simulink model "unit_can_sender"  (R2026b)
settings: Solver=FixedStepDiscrete  FixedStep=0.1  EnableMultiTasking=on
values from neighbouring files (symbols this model uses):
  BOOT_SEC = 10.0    [sign_detector.sldd]
  STALL_SEC = 1.0    [sign_detector.sldd]
libraries: raspberrypiCommlib x1
settings Model: DataDictionary=sign_detector.sldd  Creator=don  LastModifiedBy=don
settings SolverCC: PositivePriorityOrder=on
settings OptimizationCC: DifferentSizesBufferReuse=on  EfficientFloat2IntCast=on  EfficientTunableParamExpr=on  EnhancedBackFolding=on  LifeSpan=Inf  MaxStackSize=200000  OptimizationCustomize=off  OptimizeBlockOrder=speed  PassReuseOutputArgsAs=Individual arguments  UseDivisionForNetSlopeComputation=on
settings DebuggingCC: AlgebraicLoopMsg=error  ArtificialAlgebraicLoopMsg=error  AssertControl=DisableAll  BlockPriorityViolationMsg=error  BusObjectLabelMismatch=error  CheckMatrixSingularityMsg=error  InheritedTsInSrcMsg=error  IntegerOverflowMsg=error  IntegerSaturationMsg=error  ModelReferenceDataLoggingMessage=error  ModelReferenceIOMismatchMessage=error  NonBusSignalsTreatedAsBus=error  ParameterPrecisionLossMsg=error  ParameterTunabilityLossMsg=error  ParameterUnderflowMsg=error  ReadBeforeWriteMsg=EnableAllAsError  RootOutportRequireBusObject=error  SFcnCompatibilityMsg=error  SaveWithDisabledLinksMsg=error  SaveWithParameterizedLinksMsg=error  SigSpecEnsureSampleTimeMsg=error  SignalInfNanChecking=error  SignalLabelMismatchMsg=error  SignalRangeChecking=error  SolverPrmCheckMsg=error  StateNameClashWarn=warning  StrictBusMsg=ErrorOnBusTreatedAsVector  TasksWithSamePriorityMsg=error  UnconnectedInputMsg=error  UnconnectedLineMsg=error  UnconnectedOutputMsg=error  UnderSpecifiedDataTypeMsg=error  UniqueDataStoreMsg=error  UnknownTsInhSupMsg=error  UnnecessaryDatatypeConvMsg=warning  VariantConditionMismatch=error  VectorMatrixConversionMsg=error  WriteAfterReadMsg=EnableAllAsError  WriteAfterWriteMsg=EnableAllAsError
settings HardwareCC: ProdHWDeviceType=ARM Compatible->ARM Cortex-A (64-bit)  ProdLargestAtomicFloat=Double  ProdLargestAtomicInteger=LongLong  ProdLongLongMode=on
settings ModelReferenceCC: ModelReferenceNumInstancesAllowed=Single
settings SFSimCC: EnableRuntimeRecursion=off  MATLABDynamicMemAlloc=off
settings RTWCC: BuildConfiguration=Faster Runs  Description=Embedded Coder  HardwareBoard=Raspberry Pi (64bit)  SystemTargetFile=ert.tlc  TLCOptions="-aInlineSetEventsForThisBaseRateFcn=TLC_FALSE -aSuppressMultiTaskScheduler=TLC_FALSE  -aRateBasedStepFcn=0"  TargetLang=C++  TemplateMakefile=ert_default_tmf  Toolchain=GNU GCC RPIUtils
settings CodeAppCC: ForceParamTrailComments=on  IgnoreCustomStorageClasses=off  InsertBlockDesc=on  MATLABFcnDesc=on  MATLABSourceComments=on  OperatorAnnotations=on  ReqsInCode=on  SFDataObjDesc=on  SimulinkDataObjDesc=on  StateflowObjectComments=on
settings ERTTargetCC: CastingMode=Standards  CombineSignalStateStructs=on  EnableSignedLeftShifts=off  EnableSignedRightShifts=off  ExtModeIntrfLevel=Level2 - Open  ExtModeMexFile=ext_xcp  ExtModeStaticAlloc=on  GenerateSharedConstants=off  ParenthesesLevel=Standards  PreserveExpressionOrder=on  SubcomponentCodeInterfacePackaging=Nonreusable function  SupportNonFinite=off  SupportVariableSizeSignals=on  SuppressErrorStatus=on  TargetLangStandard=C++11 (ISO)  UtilityFuncGeneration=Shared location

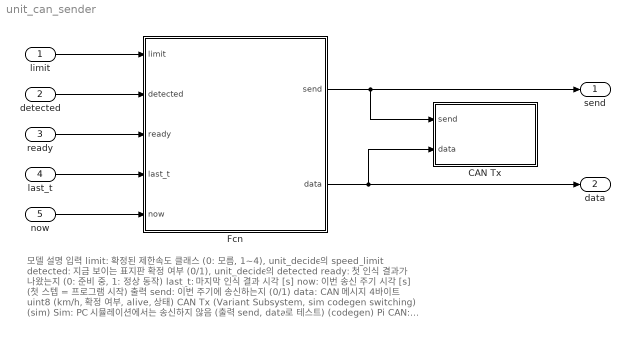
== system unit_can_sender ==
  note: 모델 설명
      | 입력
      | limit: 확정된 제한속도 클래스 (0: 모름, 1~4), unit_decide의 speed_limit
      | detected: 지금 보이는 표지판 확정 여부 (0/1), unit_decide의 detected
      | ready: 첫 인식 결과가 나왔는지 (0: 준비 중, 1: 정상 동작)
      | last_t: 마지막 인식 결과 시각 [s]
      | now: 이번 송신 주기 시각 [s] (첫 스텝 = 프로그램 시작)
      | 출력
      | send: 이번 주기에 송신하는지 (0/1)
      | data: CAN 메시지 4바이트 uint8 (km/h, 확정 여부, alive, 상태)
      | CAN Tx (Variant Subsystem, sim codegen switching)
      | (sim) Sim: PC 시뮬레이션에서는 송신하지 않음 (출력 send, data로 테스트)
      | (codegen) Pi CAN: send = 1인 주기에 Raspberry Pi CAN Transmit으로 송신
      | can0, ID 0x100(256), 표준 ID, 4바이트, Raw data, 기다리지 않음
      | can0이 다시 준비되면 자동 재개 (SWR-33), can0 설정은 OS에서 (SWR-35)
  limit : Inport  OutDataTypeStr=double  PortDimensions=1  Interpolate=off
  detected : Inport  Port=2  OutDataTypeStr=double  PortDimensions=1  Interpolate=off
  ready : Inport  Port=3  OutDataTypeStr=double  PortDimensions=1  Interpolate=off
  last_t : Inport  Port=4  OutDataTypeStr=double  PortDimensions=1  Interpolate=off
  now : Inport  Port=5  OutDataTypeStr=double  PortDimensions=1  Interpolate=off
  CAN Tx : Subsystem  Variant=on  VariantControlMode=sim codegen switching
  Fcn : MATLAB Function  TreatAsAtomicUnit=on
  send : Outport
  data : Outport  Port=2
  wires:
  limit/1 -> Fcn/1(limit)
  detected/1 -> Fcn/2(detected)
  ready/1 -> Fcn/3(ready)
  last_t/1 -> Fcn/4(last_t)
  now/1 -> Fcn/5(now)
  Fcn/1(send) -> send/1, CAN Tx/1(send)
  Fcn/2(data) -> data/1, CAN Tx/2(data)

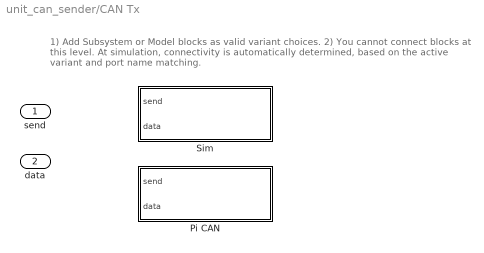
== system unit_can_sender/CAN Tx ==
  note: 1) Add Subsystem or Model blocks as valid variant choices.
      | 2) You cannot connect blocks at this level. At simulation, connectivity is automatically
      | determined, based on the active variant and port name matching.
  send : Inport
  data : Inport  Port=2
  Pi CAN : Subsystem  VariantControl=(codegen)
  Sim : Subsystem  VariantControl=(sim)

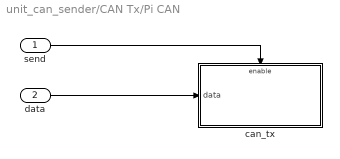
== system unit_can_sender/CAN Tx/Pi CAN ==
  send : Inport
  data : Inport  Port=2
  can_tx : Subsystem  TreatAsAtomicUnit=on
  wires:
  send/1 -> can_tx/Enable
  data/1 -> can_tx/1(data)

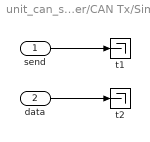
== system unit_can_sender/CAN Tx/Sim ==
  send : Inport
  data : Inport  Port=2
  t1 : Terminator
  t2 : Terminator
  wires:
  send/1 -> t1/1
  data/1 -> t2/1

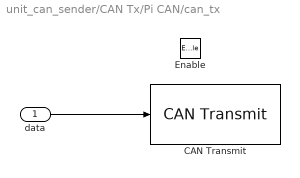
== system unit_can_sender/CAN Tx/Pi CAN/can_tx ==
  data : Inport
  Enable : EnablePort
  CAN Transmit : raspberrypiCommlib/CAN Transmit  DeviceID=can0  SetupCAN=off  TypeofCAN=Real  InputDataType=Raw data  BlockingMode_=off  BlockTimeout_=1  OutputStatus=off  IdentifierType=Standard (11-bit identifier)  MessageId=256  MsgLength=4  RemoteFrame=off  SimulateUsing=Code generation
  wires:
  data/1 -> CAN Transmit/1

== matlab function unit_can_sender/Fcn ==
  data: limit input double; send output double; detected input double; ready input double; last_t input double; now input double; data output uint8 size=[4 1]; STALL_SEC parameter double; BOOT_SEC parameter double
function [send, data] = can_sender(limit, detected, ready, last_t, now, STALL_SEC, BOOT_SEC)

TOL = 1e-9; % 시각 비교 오차 [초] (소수 합의 반올림 오차 보정)
KMH = uint8([0 30 60 90 120]); % 클래스값 0~4 -> km/h (SWR-11 byte0)

persistent alive start_t
if isempty(alive)
    alive = uint8(0);  % 다음 메시지의 alive counter
    start_t = now;     % 프로그램 시작 시각 (SWR-34의 BOOT_SEC 기준)
end

% 송신 여부
if ready == 1
    send = double(now - last_t < STALL_SEC - TOL);
else
    send = double(now - start_t < BOOT_SEC - TOL);
end

% 메시지 (송신하지 않는 주기에도 만들어 둠)
data = zeros(4, 1, 'uint8');
if limit >= 0 && limit <= 4 && limit == floor(limit)
    data(1) = KMH(limit + 1);
end
if detected == 0 || detected == 1
    data(2) = uint8(detected);
end
data(3) = alive;
if ready == 0 || ready == 1
    data(4) = uint8(ready);
end

% alive counter 증가 (uint8 포화를 피하려고 255 다음 0을 직접 처리)
if send == 1
    if alive == uint8(255)
        alive = uint8(0);
    else
        alive = alive + uint8(1);
    end
end
end
